simulink model "motor_sim_impairments"  (R2013b)
settings: Solver=ode45  StartTime=0.0  StopTime=Tsim_final  FixedStep=sim_step_size  RelTol=1e-3
values from neighbouring files (symbols this model uses):
  b = 0.01    [motor_parameters.m]    (also in motor_simulation_run.m = 0)
  J = 0.002    [motor_parameters.m]
  Kb = 0.7    [motor_parameters.m]
  Kt = 0.7    [motor_parameters.m]
  R = 10    [motor_parameters.m]
  RAD2Counts = 720/(2*pi)    (= 114.591559026)    [motor_parameters.m]
  sim_step_size = TS    (= 0.015)    [motor_sim_impairments_run.m]    (also in motor_simulation_run.m = 0.0001)
  TS = 0.015    [motor_sim_impairments_run.m]
  Vsupply = 4.5    [motor_parameters.m]
libraries: simulink x1
settings Model: Creator=nding  LastModifiedBy=nding

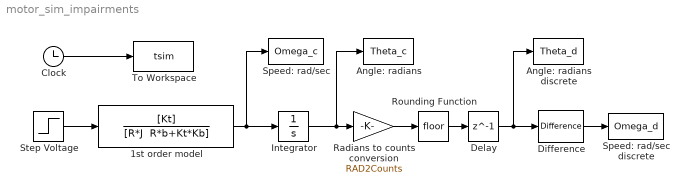
== system motor_sim_impairments ==
  1st order model : TransferFcn  Numerator=[Kt]  Denominator="[R*J  R*b+Kt*Kb]"
  Angle: radians : ToWorkspace  VariableName=Theta_c  SampleTime=sim_step_size
  Angle: radians discrete : ToWorkspace  VariableName=Theta_d  SampleTime=sim_step_size
  Clock : Clock
  Delay : Delay  DelayLength=1  SampleTime=TS
  Difference : simulink/Discrete/Difference  ICPrevInput=0.0  InputProcessing=Inherited  OutMin=[]  OutMax=[]  OutDataType=fixdt(1, 16)  OutScaling=2^-10  DoSatur=off
  Integrator : Integrator
  Radians to counts conversion : Gain  Gain=RAD2Counts
  Rounding Function : Rounding
  "Speed: rad/sec " : ToWorkspace  VariableName=Omega_c  SampleTime=sim_step_size
  Speed: rad/sec discrete : ToWorkspace  VariableName=Omega_d  SampleTime=sim_step_size
  Step Voltage : Step  Time=0  After=Vsupply  SampleTime=0
  To Workspace : ToWorkspace  VariableName=tsim  SampleTime=sim_step_size
  wires:
  Clock/1 -> To Workspace/1
  Step Voltage/1 -> 1st order model/1
  1st order model/1 -> Integrator/1, "Speed: rad/sec "/1
  Integrator/1 -> Angle: radians/1, Radians to counts conversion/1
  Radians to counts conversion/1 -> Rounding Function/1
  Delay/1 -> Angle: radians discrete/1, Difference/1
  Difference/1 -> Speed: rad/sec discrete/1
  Rounding Function/1 -> Delay/1
